simulink model "Full_Wave_Center_Tapped"  (R2025b)
settings: Solver=VariableStepAuto  StartTime=0.0  StopTime=10.0  MaxStep=1e-4  RelTol=1e-3
undefined symbols (not defined in the file): b42f625b
libraries: fl_lib x13, nesl_utility x7, ee_lib x2
settings Model: Creator=USER  LastModifiedBy=USER

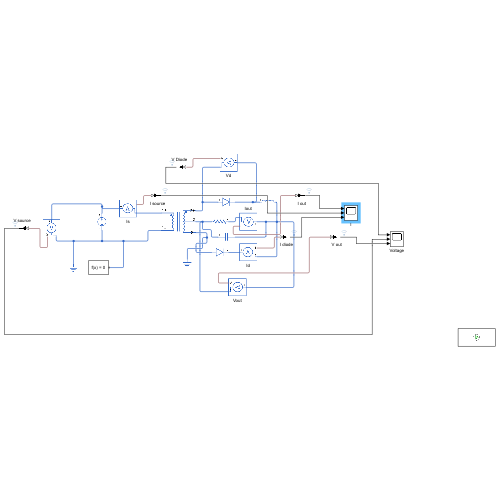
[thumbnail: Simulink's stored preview of the top-level diagram]
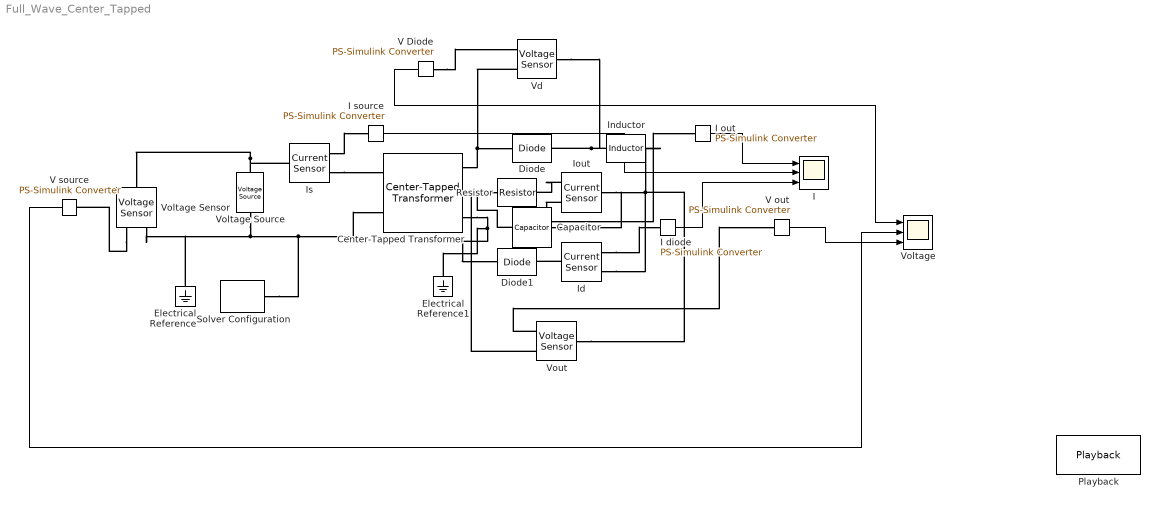
== system Full_Wave_Center_Tapped ==
  Capacitor : fl_lib/Electrical/Electrical Elements/Capacitor  c=200e-6 F  r=1e-6 Ohm  g=0 1/Ohm  i_specify=off  i_priority=None  i=0 A  i_nominal_specify=off  i_nominal_value=1  i_nominal_unit=A  v_specify=off  v_priority=None  v=0 V  v_nominal_specify=off  v_nominal_value=1  v_nominal_unit=V  vc_specify=off  vc_priority=High  vc=0 V  vc_nominal_specify=off  vc_nominal_value=1  vc_nominal_unit=V
  Center-Tapped Transformer : ee_lib/Passive/Transformers/Center-Tapped Transformer  modeling_option=ee.enum.transformer_option.ideal  n=1  T=0.5  Rw1=0.01 Ohm  L1=0.0001 H  Rw2=0.01 Ohm  L2=0.0001 H  Rm=100 Ohm  Lm=0.04 H  i1_specify=off  i1_priority=None  i1=0 A  i1_nominal_specify=off  i1_nominal_value=1  i1_nominal_unit=A  i2p_specify=off  i2p_priority=None  i2p=0 A  i2p_nominal_specify=off  i2p_nominal_value=1  i2p_nominal_unit=A  i2n_specify=off  i2n_priority=None  i2n=0 A  i2n_nominal_specify=off  i2n_nominal_value=1  i2n_nominal_unit=A
      settings: InternalSimscapePortConfiguration="{\"Bottom\":[],\"Left\":[{\"id\":\"p1\",\"label\":\"1+\",\"type\":\"foundation.electrical.electrical\"},{\"id\":\"n1\",\"label\":\"1-\",\"type\":\"foundation.electrical.electrical\"}],\"Right\":[{\"id\":\"p2\",\"label\":\"2+\",\"type\":\"foundation.electrical.electrical\"},{\"id\":\"c\",\"label\":\"c\",\"type\":\"foundation.electrical.electrical\"},{\"id\":\"n2\",\"label\":\"2-\",\"type\":\"foundation.electrical.electrical\"}],\"Top\":[]}"
  Diode : fl_lib/Electrical/Electrical Elements/Diode  Vf=0.6 V  Ron=0.3 Ohm  Goff=1e-8 1/Ohm  i_specify=off  i_priority=None  i=0 A  i_nominal_specify=off  i_nominal_value=1  i_nominal_unit=A  v_specify=off  v_priority=None  v=0 V  v_nominal_specify=off  v_nominal_value=1  v_nominal_unit=V
  Diode1 : fl_lib/Electrical/Electrical Elements/Diode  Vf=0.6 V  Ron=0.3 Ohm  Goff=1e-8 1/Ohm  i_specify=off  i_priority=None  i=0 A  i_nominal_specify=off  i_nominal_value=1  i_nominal_unit=A  v_specify=off  v_priority=None  v=0 V  v_nominal_specify=off  v_nominal_value=1  v_nominal_unit=V
  Electrical Reference : fl_lib/Electrical/Electrical Elements/Electrical Reference
  Electrical Reference1 : fl_lib/Electrical/Electrical Elements/Electrical Reference
  I : Scope  NumInputPorts=3
      settings: ActiveDisplayYMinimum=-2.7003409599285488  ActiveDisplayYMaximum=4.6642245193575773  DataLoggingVariableName=ScopeData4
  I diode : nesl_utility/PS-Simulink Converter  PhysicalDomain=network_engine_domain  SubClassName=ps_output  LeftPortType=input  RightPortType=output  PseudoPeriodic=off  Frequencies=[]  VectorFormat=inherit  Unit=inherit  AffineConversion=off
  I out : nesl_utility/PS-Simulink Converter  PhysicalDomain=network_engine_domain  SubClassName=ps_output  LeftPortType=input  RightPortType=output  PseudoPeriodic=off  Frequencies=[]  VectorFormat=inherit  Unit=inherit  AffineConversion=off
  I source : nesl_utility/PS-Simulink Converter  PhysicalDomain=network_engine_domain  SubClassName=ps_output  LeftPortType=input  RightPortType=output  PseudoPeriodic=off  Frequencies=[]  VectorFormat=inherit  Unit=inherit  AffineConversion=off
  Id : fl_lib/Electrical/Electrical Sensors/Current Sensor
  Inductor : fl_lib/Electrical/Electrical Elements/Inductor  l=120 mH  r=0 Ohm  g=1e-9 1/Ohm  i_specify=off  i_priority=None  i=0 A  i_nominal_specify=off  i_nominal_value=1  i_nominal_unit=A  v_specify=off  v_priority=None  v=0 V  v_nominal_specify=off  v_nominal_value=1  v_nominal_unit=V  i_L_specify=off  i_L_priority=High  i_L=0 A  i_L_nominal_specify=off  i_L_nominal_value=1  i_L_nominal_unit=A
  Iout : fl_lib/Electrical/Electrical Sensors/Current Sensor
  Is : fl_lib/Electrical/Electrical Sensors/Current Sensor
  Playback : Playback  NumPorts=0  PartName=b42f625b-4ccf-4a7a-8c84-3c7dab1f01fb  TablePosition=Bottom
  Resistor : fl_lib/Electrical/Electrical Elements/Resistor  R=100 Ohm  i_specify=off  i_priority=None  i=0 A  i_nominal_specify=off  i_nominal_value=1  i_nominal_unit=A  v_specify=off  v_priority=None  v=0 V  v_nominal_specify=off  v_nominal_value=1  v_nominal_unit=V
  Solver Configuration : nesl_utility/Solver Configuration  PhysicalDomain=network_engine_domain  SubClassName=solver  LeftPortType=input  RightPortType=generic  Tones=[]  Harmonics=[]  SimulateNoise=off  Profile=off  UseLocalSampling=off  EnableSwitchedLinearOptims=on  FrequencyDomain=off  UseCCode=off  RelTol=0.001  AbsTol=0.001  MinStep=1e-09  ToWorkspace=off  RevertToSquareIcSolve=off  NumHomotopyIterations=100  PhasorMode=off  PhasorModeNumHarmonics=1  ConsistencySolver=NEWTON_XTOL_AFTER_FTOL  IndexReductionMethod=DerivativeReplacement  DoDC=off  ResidualTolerance=1e-09  ConsistencyTolSource=GLOBAL  ConsistencyAbsTol=0.001  ConsistencyRelTol=0.001  ConsistencyTolFactor=0.001  UseLocalSolver=off  LocalSolverChoice=NE_BACKWARD_EULER_ADVANCER  ResolveIndetEquations=on  FunctionEvalNumThread=1  LocalSolverSampleTime=0.001  DoFixedCost=off  MaxNonlinIter=3  MaxModeIter=2  ComputeImpulses=off  ImpulseIterations=2  LinearAlgebra=auto  LinearAlgebraNumThread=0  EquationFormulation=NE_TIME_EF  DelaysMemoryBudget=1024  AutomaticFiltering=on  FilteringTimeConstant=0.001  PartitionStorageMethod=AS_NEEDED  PartitionMemoryBudget=1024  PartitionMethod=ROBUST  MultibodyUseLocalSolver=off  MultibodyLocalSolverChoice=ODE1  MultibodyLocalSolverSampleTime=0.001
  V Diode : nesl_utility/PS-Simulink Converter  PhysicalDomain=network_engine_domain  SubClassName=ps_output  LeftPortType=input  RightPortType=output  PseudoPeriodic=off  Frequencies=[]  VectorFormat=inherit  Unit=inherit  AffineConversion=off
  V out : nesl_utility/PS-Simulink Converter  PhysicalDomain=network_engine_domain  SubClassName=ps_output  LeftPortType=input  RightPortType=output  PseudoPeriodic=off  Frequencies=[]  VectorFormat=inherit  Unit=inherit  AffineConversion=off
  V source : nesl_utility/PS-Simulink Converter  PhysicalDomain=network_engine_domain  SubClassName=ps_output  LeftPortType=input  RightPortType=output  PseudoPeriodic=off  Frequencies=[]  VectorFormat=inherit  Unit=inherit  AffineConversion=off
  Vd : fl_lib/Electrical/Electrical Sensors/Voltage Sensor
  Voltage : Scope  NumInputPorts=3
      settings: ActiveDisplayYMinimum=-159.07068455059243  ActiveDisplayYMaximum=159.06827226812214
  Voltage Sensor : fl_lib/Electrical/Electrical Sensors/Voltage Sensor
  Voltage Source : ee_lib/Sources/Voltage Source  dc_voltage=0 V  ac_voltage=127.27 V  ac_shift=0 rad  ac_frequency=60 Hz  noise_mode=ee.enum.sources.noise.Disabled  PSD=0 V^2/Hz  sample_time=1e-3 s  repeatability=ee.enum.sources.repeatability.NotRepeatable  user_seed=0  auto_seed=3499211588  i_specify=off  i_priority=None  i=0 A  i_nominal_specify=off  i_nominal_value=1  i_nominal_unit=A  v_specify=off  v_priority=None  v=0 V  v_nominal_specify=off  v_nominal_value=1  v_nominal_unit=V
  Vout : fl_lib/Electrical/Electrical Sensors/Voltage Sensor
  wires:
  V out/1 -> Voltage/3
  V source/1 -> Voltage/2
  V Diode/1 -> Voltage/1
  I diode/1 -> I/3
  I out/1 -> I/1
  I source/1 -> I/2
  connections:
  Voltage Source/LConn1 -- Is/LConn1 -- Voltage Sensor/LConn1
  Voltage Source/RConn1 -- Electrical Reference/LConn1 -- Voltage Sensor/RConn2 -- Solver Configuration/RConn1 -- Center-Tapped Transformer/LConn2
  Center-Tapped Transformer/RConn2 -- Capacitor/LConn1 -- Resistor/LConn1 -- Vout/RConn2
  Center-Tapped Transformer/RConn3 -- Electrical Reference1/LConn1 -- Diode1/LConn1
  Center-Tapped Transformer/RConn1 -- Vd/RConn2 -- Diode/LConn1
  Vout/LConn1 -- Capacitor/RConn1 -- Iout/LConn1 -- Inductor/RConn1 -- Id/RConn2
  Vout/RConn1 -- V out/LConn1
  Voltage Sensor/RConn1 -- V source/LConn1
  Is/RConn2 -- Center-Tapped Transformer/LConn1
  V Diode/LConn1 -- Vd/RConn1
  Is/RConn1 -- I source/LConn1
  Id/LConn1 -- Diode1/RConn1
  Id/RConn1 -- I diode/LConn1
  Iout/RConn1 -- I out/LConn1
  Iout/RConn2 -- Resistor/RConn1
  Vd/LConn1 -- Inductor/LConn1 -- Diode/RConn1
